simulink model "powertrain_model"  (R2025a)
settings: Solver=ode23tb  StartTime=0.0  StopTime=simlength  FixedStep=tc  MaxStep=tc
values from neighbouring files (symbols this model uses):
  angle_error = angle_error_deg/180*pi    (= 0)    [init_model.m]
  CTRPIFF_CLIP_RELEASE = 0.001    [init_model.m]
  dead_time = dead_time_INV    (= 4.2e-07)    [init_model.m]
  dead_time_INV = 0.42e-6    (= 4.2e-07)    [init_model.m]
  DThs_init = 0    [init_model.m]
  emf_fb_p = 0.2    [init_model.m]
  emf_fb_p_ccaller_1 = emf_fb_p    (= 0.2)    [init_model.m]
  emf_fb_p_ccaller_2 = emf_fb_p    (= 0.2)    [init_model.m]
  emf_p = emf_fb_p*4/10    (= 0.08)    [init_model.m]
  emf_p_ccaller_1 = emf_fb_p_ccaller_1*4/10    (= 0.08)    [init_model.m]
  emf_p_ccaller_2 = emf_fb_p_ccaller_2*4/10    (= 0.08)    [init_model.m]
  fPWM_INV = 25e3    (= 25000)    [init_model.m]
  g0_reference_flt = fcut_reference_flt * ts_inv * 2*pi    (= 0.00100530964915)    [init_model.m]
  g1_reference_flt = 1 - g0_reference_flt    (= 0.998994690351)    [init_model.m]
  id_ref_if_pu = iload_rms_ref*sqrt(2)/ibez    [init_model.m]
  kalman_omega = kw    [init_model.m]
  kalman_theta = kg    [init_model.m]
  kg = K(1)    [init_model.m]
  ki_id = 2    [analysis_cc.m]    (also in init_model.m = 9)
  ki_iq = 9    [init_model.m]
  ki_w = 1    [init_model.m]
  kp_id = 0.15    [analysis_cc.m]    (also in init_model.m = 0.25)
  kp_iq = 0.2    [init_model.m]
  kp_w = 1    [init_model.m]
  kw = K(2)    [init_model.m]
  luenberger_l1 = Klo(1)    [init_model.m]
  luenberger_l2 = Klo(2)    [init_model.m]
  luenberger_l3 = Klo(3)    [init_model.m]
  motorc_m_scale = 2/3*Vdc_bez/ubez    [init_model.m]
  number_of_cells = 100    [init_model.m]
  omega_flt_fcut = 10    [init_model.m]
  omega_flt_g0 = omega_flt_fcut * ts_inv * 2*pi    (= 0.00251327412287)    [init_model.m]
  omega_flt_g1 = 1 - omega_flt_g0    (= 0.997486725877)    [init_model.m]
  omega_ref_if_pu = 1200*2*pi/omega_bez    [init_model.m]
  phase_compensation_omega = 0    [init_model.m]
  pwm_out_lim = 1    [init_model.m]
  Q = 10    [init_model.m]
  q1Kalman = ts_inv^2    (= 1.6e-09)    [init_model.m]
  q2Kalman = ts_inv^1    (= 4e-05)    [init_model.m]
  q3Kalman = 0    [init_model.m]
  rKalman = 1    [init_model.m]
  Tambient = 1    [init_model.m]
  tc = ts_inv/200    (= 2e-07)    [init_model.m]
  time_init = 0.025    [init_model.m]
  torque_ref = 64/ibez*torque_mode    [init_model.m]
  ts_inv = 1/fPWM_INV    (= 4e-05)    [init_model.m]
  tsample = ts_inv    (= 4e-05)    [init_model.m]
  u_flt_g0 = u_flt_fcut * ts_inv * 2*pi    (= 0.904778684234)    [init_model.m]
  u_flt_g1 = 1 - u_flt_g0    (= 0.0952213157661)    [init_model.m]
  Vdc_bez = 400    [init_model.m]
undefined symbols (not defined in the file or in its folder): b, ibez, Jm, Jm_norm, Ld_norm, Lq_norm, Ls_norm, magnitude, omega_bez, psi_bez, psi_m, psi_m_norm, R_RLload, Rload_eq, Rs_norm, tau_bez, weigth
libraries: fl_lib x100, nesl_utility x84, ee_lib x11, cstblocks x4, lithium_ion_cell_lib x1, simulink x1, pmsm_uvw_with_harmonics_lib x1, pmsm_spatial_harmonics_uvw_lib x1, flexshaft_lib x1
(part 3 of 6)

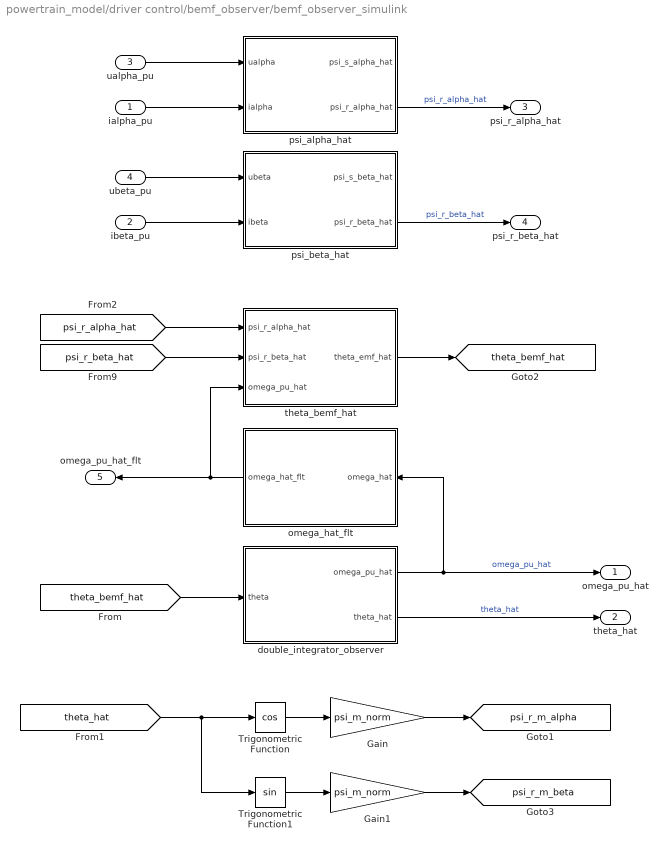
== system powertrain_model/driver control/bemf_observer/bemf_observer_simulink ==
  ialpha_pu : Inport
  ibeta_pu : Inport  Port=2
  ualpha_pu : Inport  Port=3
  ubeta_pu : Inport  Port=4
  Gain : Gain  Gain=psi_m_norm
  Gain1 : Gain  Gain=psi_m_norm
  Trigonometric Function : Trigonometry  Operator=cos
  Trigonometric Function1 : Trigonometry
  double_integrator_observer : Subsystem
  omega_hat_flt : Subsystem
  psi_alpha_hat : Subsystem
  psi_beta_hat : Subsystem
  theta_bemf_hat : Subsystem
  omega_pu_hat : Outport
  theta_hat : Outport  Port=2
  psi_r_alpha_hat : Outport  Port=3
  psi_r_beta_hat : Outport  Port=4
  omega_pu_hat_flt : Outport  Port=5
  tag scope: psi_r_m_alpha=global, psi_r_m_beta=global, theta_bemf_hat=global
  wires:
  omega_hat_flt/1(omega_hat_flt) -> omega_pu_hat_flt/1, theta_bemf_hat/3(omega_pu_hat)
  psi_alpha_hat/2(psi_r_alpha_hat) -> psi_r_alpha_hat/1  "psi_r_alpha_hat"
  double_integrator_observer/1(omega_pu_hat) -> omega_pu_hat/1, omega_hat_flt/1(omega_hat)  "omega_pu_hat"
  double_integrator_observer/2(theta_hat) -> theta_hat/1  "theta_hat"
  psi_beta_hat/2(psi_r_beta_hat) -> psi_r_beta_hat/1  "psi_r_beta_hat"
  [theta_bemf_hat] -> double_integrator_observer/1(theta)
  theta_bemf_hat/1(theta_emf_hat) -> [theta_bemf_hat]
  Gain1/1 -> [psi_r_m_beta]
  Gain/1 -> [psi_r_m_alpha]
  [theta_hat] -> Trigonometric Function1/1, Trigonometric Function/1
  ubeta_pu/1 -> psi_beta_hat/1(ubeta)
  ualpha_pu/1 -> psi_alpha_hat/1(ualpha)
  ibeta_pu/1 -> psi_beta_hat/2(ibeta)
  ialpha_pu/1 -> psi_alpha_hat/2(ialpha)
  Trigonometric Function1/1 -> Gain1/1
  Trigonometric Function/1 -> Gain/1
  [psi_r_alpha_hat] -> theta_bemf_hat/1(psi_r_alpha_hat)
  [psi_r_beta_hat] -> theta_bemf_hat/2(psi_r_beta_hat)

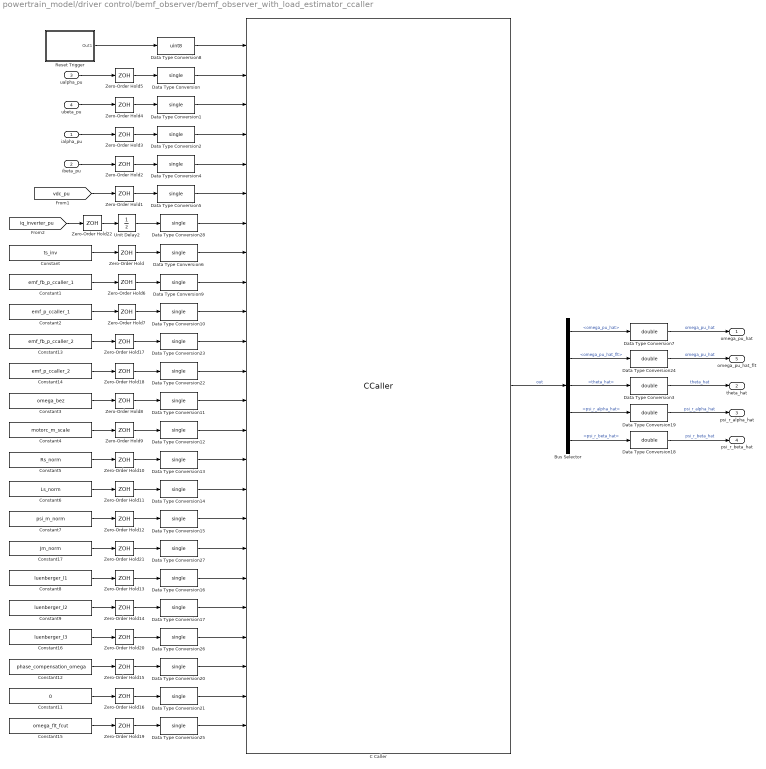
== system powertrain_model/driver control/bemf_observer/bemf_observer_with_load_estimator_ccaller ==
  ialpha_pu : Inport
  ibeta_pu : Inport  Port=2
  ualpha_pu : Inport  Port=3
  ubeta_pu : Inport  Port=4
  Bus Selector : BusSelector  OutputSignals=omega_pu_hat,omega_pu_hat_flt,theta_hat,psi_r_alpha_hat,psi_r_beta_hat
  C Caller : CCaller  FunctionName=bemf_obsv_load_est_process_simulink  PortSpecificationStruct="%)30     .    (\"P   8    (     @         %    \"    !D    !     0         %  0 \"0    $    _    07)G3F%M90  4&]R=$YA;64 4V-O<&4     26YD97@     5'EP90      4VEZ90      27-';&]B86P   X    P    !@    @    $          4    (     0    ,    !         !   P!O=70 #@   #     &    \"     0         !0    @    !     P    $         $  # &]U=  .    .     8    (    !          %    \"     $    &     0         0  ...(+14838 chars)"  SampleTime=ts_inv
  Constant : Constant  Value=ts_inv
  Constant1 : Constant  Value=emf_fb_p_ccaller_1
  Constant11 : Constant  Value=0
  Constant12 : Constant  Value=phase_compensation_omega  VectorParams1D=off
  Constant13 : Constant  Value=emf_fb_p_ccaller_2
  Constant14 : Constant  Value=emf_p_ccaller_2
  Constant15 : Constant  Value=omega_flt_fcut
  Constant16 : Constant  Value=luenberger_l3
  Constant17 : Constant  Value=Jm_norm
  Constant2 : Constant  Value=emf_p_ccaller_1
  Constant3 : Constant  Value=omega_bez
  Constant4 : Constant  Value=motorc_m_scale
  Constant5 : Constant  Value=Rs_norm
  Constant6 : Constant  Value=Ls_norm
  Constant7 : Constant  Value=psi_m_norm
  Constant8 : Constant  Value=luenberger_l1
  Constant9 : Constant  Value=luenberger_l2
  Data Type Conversion{,1..2,4..6,9..17,20..23,25..28} (23 alike) : DataTypeConversion  OutDataTypeStr=single  SaturateOnIntegerOverflow=off  RndMeth=Floor
  Data Type Conversion{3,7,18..19,24} (5 alike) : DataTypeConversion  OutDataTypeStr=double  SaturateOnIntegerOverflow=off  RndMeth=Floor
  Data Type Conversion8 : DataTypeConversion  OutDataTypeStr=uint8  SaturateOnIntegerOverflow=off  RndMeth=Floor
  Reset Trigger : Subsystem
  Unit Delay2 : UnitDelay  SampleTime=ts_inv  HasFrameUpgradeWarning=on
  Zero-Order Hold{,1..22} (23 alike) : ZeroOrderHold  SampleTime=ts_inv
  omega_pu_hat : Outport
  theta_hat : Outport  Port=2
  psi_r_alpha_hat : Outport  Port=3
  psi_r_beta_hat : Outport  Port=4
  omega_pu_hat_flt : Outport  Port=5
  wires:
  Data Type Conversion5/1 -> C Caller/6
  Data Type Conversion/1 -> C Caller/2
  Data Type Conversion1/1 -> C Caller/3
  Data Type Conversion4/1 -> C Caller/5
  Data Type Conversion2/1 -> C Caller/4
  Zero-Order Hold/1 -> Data Type Conversion6/1
  Zero-Order Hold5/1 -> Data Type Conversion/1
  Zero-Order Hold4/1 -> Data Type Conversion1/1
  Zero-Order Hold3/1 -> Data Type Conversion2/1
  Zero-Order Hold2/1 -> Data Type Conversion4/1
  Zero-Order Hold1/1 -> Data Type Conversion5/1
  [vdc_pu] -> Zero-Order Hold1/1
  Constant/1 -> Zero-Order Hold/1
  ualpha_pu/1 -> Zero-Order Hold5/1
  ialpha_pu/1 -> Zero-Order Hold3/1
  ubeta_pu/1 -> Zero-Order Hold4/1
  ibeta_pu/1 -> Zero-Order Hold2/1
  Reset Trigger/1(Out1) -> Data Type Conversion8/1
  Data Type Conversion8/1 -> C Caller/1
  Zero-Order Hold6/1 -> Data Type Conversion9/1
  Zero-Order Hold7/1 -> Data Type Conversion10/1
  Zero-Order Hold8/1 -> Data Type Conversion11/1
  Zero-Order Hold9/1 -> Data Type Conversion12/1
  Zero-Order Hold10/1 -> Data Type Conversion13/1
  Zero-Order Hold11/1 -> Data Type Conversion14/1
  Zero-Order Hold12/1 -> Data Type Conversion15/1
  Zero-Order Hold13/1 -> Data Type Conversion16/1
  Zero-Order Hold14/1 -> Data Type Conversion17/1
  Constant3/1 -> Zero-Order Hold8/1
  Constant4/1 -> Zero-Order Hold9/1
  Constant5/1 -> Zero-Order Hold10/1
  Constant8/1 -> Zero-Order Hold13/1
  Constant9/1 -> Zero-Order Hold14/1
  Constant6/1 -> Zero-Order Hold11/1
  Constant7/1 -> Zero-Order Hold12/1
  C Caller/1 -> Bus Selector/1  "out"
  Data Type Conversion7/1 -> omega_pu_hat/1  "omega_pu_hat"
  Data Type Conversion3/1 -> theta_hat/1  "theta_hat"
  Data Type Conversion19/1 -> psi_r_alpha_hat/1  "psi_r_alpha_hat"
  Data Type Conversion18/1 -> psi_r_beta_hat/1  "psi_r_beta_hat"
  Constant1/1 -> Zero-Order Hold6/1
  Constant2/1 -> Zero-Order Hold7/1
  Constant12/1 -> Zero-Order Hold15/1
  Zero-Order Hold15/1 -> Data Type Conversion20/1
  Zero-Order Hold16/1 -> Data Type Conversion21/1
  Constant11/1 -> Zero-Order Hold16/1
  Constant14/1 -> Zero-Order Hold18/1
  Constant13/1 -> Zero-Order Hold17/1
  Zero-Order Hold18/1 -> Data Type Conversion22/1
  Zero-Order Hold17/1 -> Data Type Conversion23/1
  Data Type Conversion24/1 -> omega_pu_hat_flt/1  "omega_pu_hat"
  Constant15/1 -> Zero-Order Hold19/1
  Zero-Order Hold19/1 -> Data Type Conversion25/1
  Bus Selector/5 -> Data Type Conversion18/1  "<psi_r_beta_hat>"
  Bus Selector/4 -> Data Type Conversion19/1  "<psi_r_alpha_hat>"
  Bus Selector/3 -> Data Type Conversion3/1  "<theta_hat>"
  Bus Selector/2 -> Data Type Conversion24/1  "<omega_pu_hat_flt>"
  Bus Selector/1 -> Data Type Conversion7/1  "<omega_pu_hat>"
  Constant16/1 -> Zero-Order Hold20/1
  Zero-Order Hold20/1 -> Data Type Conversion26/1
  Constant17/1 -> Zero-Order Hold21/1
  Zero-Order Hold21/1 -> Data Type Conversion27/1
  Data Type Conversion6/1 -> C Caller/8
  Data Type Conversion9/1 -> C Caller/9
  Data Type Conversion10/1 -> C Caller/10
  Data Type Conversion23/1 -> C Caller/11
  Data Type Conversion22/1 -> C Caller/12
  Data Type Conversion11/1 -> C Caller/13
  Data Type Conversion12/1 -> C Caller/14
  Data Type Conversion13/1 -> C Caller/15
  Data Type Conversion14/1 -> C Caller/16
  Data Type Conversion15/1 -> C Caller/17
  Data Type Conversion27/1 -> C Caller/18
  Data Type Conversion16/1 -> C Caller/19
  Data Type Conversion17/1 -> C Caller/20
  Data Type Conversion26/1 -> C Caller/21
  Data Type Conversion20/1 -> C Caller/22
  Data Type Conversion21/1 -> C Caller/23
  Data Type Conversion25/1 -> C Caller/24
  [iq_inverter_pu] -> Zero-Order Hold22/1
  Zero-Order Hold22/1 -> Unit Delay2/1
  Data Type Conversion28/1 -> C Caller/7
  Unit Delay2/1 -> Data Type Conversion28/1

== system powertrain_model/driver control/bemf_observer/u_alpha_flt ==
  u : Inport
  Gain3 : Gain  Gain=u_flt_g1
  Gain6 : Gain  Gain=u_flt_g0
  Sum : Sum  Inputs=|++
  Unit Delay1 : UnitDelay  SampleTime=ts_inv  HasFrameUpgradeWarning=on
  u_flt : Outport  VectorParamsAs1DForOutWhenUnconnected=off
  wires:
  Sum/1 -> u_flt/1, Unit Delay1/1
  Gain3/1 -> Sum/2
  Unit Delay1/1 -> Gain3/1
  u/1 -> Gain6/1
  Gain6/1 -> Sum/1

== system powertrain_model/driver control/bemf_observer/u_beta_flt ==
  u : Inport
  Gain3 : Gain  Gain=u_flt_g1
  Gain6 : Gain  Gain=u_flt_g0
  Sum : Sum  Inputs=|++
  Unit Delay1 : UnitDelay  SampleTime=ts_inv  HasFrameUpgradeWarning=on
  u_flt : Outport  VectorParamsAs1DForOutWhenUnconnected=off
  wires:
  Gain6/1 -> Sum/1
  u/1 -> Gain6/1
  Unit Delay1/1 -> Gain3/1
  Gain3/1 -> Sum/2
  Sum/1 -> Unit Delay1/1, u_flt/1

== system powertrain_model/driver control/current_ctrl/current_transformation ==
  u : Inport
  v : Inport  Port=2
  w : Inport  Port=3
  phase : Inport  Port=4
  alphabeta2dq : MATLAB Function  TreatAsAtomicUnit=on  SystemSampleTime=ts_inv
  uvw2alphabeta : MATLAB Function  TreatAsAtomicUnit=on  SystemSampleTime=ts_inv
  tag scope: i_alpha_inverter_pu=global, i_beta_inverter_pu=global, id_inverter_pu=global, iq_inverter_pu=global
  wires:
  u/1 -> uvw2alphabeta/1(u)
  uvw2alphabeta/1(alpha) -> [i_alpha_inverter_pu], alphabeta2dq/1(alpha)  "ialpha_if_pu"
  uvw2alphabeta/2(beta) -> [i_beta_inverter_pu], alphabeta2dq/2(beta)  "ibeta_if_pu"
  v/1 -> uvw2alphabeta/2(v)
  w/1 -> uvw2alphabeta/3(w)
  alphabeta2dq/1(d) -> [id_inverter_pu]
  alphabeta2dq/2(q) -> [iq_inverter_pu]
  phase/1 -> alphabeta2dq/3(phase)

== system powertrain_model/driver control/current_ctrl/rotor_phase_selection ==
  Scope : Scope  NumInputPorts=2
      settings: ActiveDisplayYMinimum=-3.92698  ActiveDisplayYMaximum=3.92699
  Switch1 : Switch  Criteria=u2 > Threshold  Threshold=0.1  SaturateOnIntegerOverflow=off  InputSameDT=off
  Switch2 : Switch  Criteria=u2 > Threshold  Threshold=0.1  SaturateOnIntegerOverflow=off  InputSameDT=off
  Variant Source : VariantSource  VariantControls={use_gyro_model == 1, use_gyro_model == 0}
  Variant Source1 : VariantSource  VariantControls={use_I_F_control == 1, use_I_F_control == 0}
  Variant Source2 : VariantSource  VariantControls={1==0, 1==1}
  theta_ctrl : Outport
  wires:
  [omega_pu_hat] -> Switch1/2
  [theta_pmsm] -> Switch1/3
  [theta_hat] -> Switch1/1
  Switch2/1 -> Variant Source/1
  Switch1/1 -> Variant Source/2
  Variant Source/1 -> Variant Source1/2
  [theta_ref_if_control] -> Variant Source1/1
  [theta_hat] -> Switch2/1
  [theta_pmsm] -> Switch2/3
  [omega_pu_hat] -> Switch2/2
  [theta_hat] -> Variant Source2/2, Scope/2  "theta_hat"
  [theta_pmsm] -> Scope/1, Variant Source2/1  "theta_pmsm"
  [theta_hat] -> theta_ctrl/1

== system powertrain_model/driver control/current_ctrl/sample_hold_normalization ==
  iu : Inport
  iv : Inport  Port=2
  iw : Inport  Port=3
  Gain : Gain  Gain=1/ibez
  Gain1 : Gain  Gain=1/ibez
  Gain2 : Gain  Gain=1/ibez
  LTI System : cstblocks/LTI System  sys=cm_tf  IC=[]  PadeOrder=0
  LTI System1 : cstblocks/LTI System  sys=cm_tf  IC=[]  PadeOrder=0
  LTI System2 : cstblocks/LTI System  sys=cm_tf  IC=[]  PadeOrder=0
  Unit Delay : UnitDelay  SampleTime=ts_inv  HasFrameUpgradeWarning=on
  Unit Delay1 : UnitDelay  SampleTime=ts_inv  HasFrameUpgradeWarning=on
  Unit Delay4 : UnitDelay  SampleTime=ts_inv  HasFrameUpgradeWarning=on
  Zero-Order Hold : ZeroOrderHold  SampleTime=ts_inv
  Zero-Order Hold1 : ZeroOrderHold  SampleTime=ts_inv
  Zero-Order Hold2 : ZeroOrderHold  SampleTime=ts_inv
  iu_pu : Outport
  iv_pu : Outport  Port=2
  iw_pu : Outport  Port=3
  wires:
  Zero-Order Hold/1 -> Unit Delay/1
  Zero-Order Hold2/1 -> Unit Delay4/1
  Zero-Order Hold1/1 -> Unit Delay1/1
  Gain1/1 -> iv_pu/1
  Gain2/1 -> iw_pu/1
  Gain/1 -> iu_pu/1
  iu/1 -> LTI System/1
  iv/1 -> LTI System1/1
  iw/1 -> LTI System2/1
  LTI System1/1 -> Zero-Order Hold1/1
  LTI System/1 -> Zero-Order Hold/1
  LTI System2/1 -> Zero-Order Hold2/1
  Unit Delay4/1 -> Gain2/1
  Unit Delay1/1 -> Gain1/1
  Unit Delay/1 -> Gain/1

== system powertrain_model/driver control/current_ctrl/vector_current_ctrl ==
  iq_ref : Inport
  id_ref : Inport  Port=2
  MTPA : Subsystem
      settings: PortSchema="{\"entries\":[{\"content\":{\"sides\":[{\"content\":{\"connectorIds\":[\"In1\"]},\"type\":\"ConnectorPlacement.EquallySpacedRectSide\",\"uuid\":\"b7b50820-32cf-4b06-b710-c36db40508fb\"},{\"content\":{\"connectorIds\":[\"Out1\"],\"side\":\"RIGHT\"},\"type\":\"ConnectorPlacement.EquallySpacedRectSide\",\"uuid\":\"9680176d-6365-4ae4-8330-83815ae14f93\"},{\"content\":{\"connectorIds\":[\"In2\"],\"side\":\"TOP\"},\"type\":\"ConnectorPlacement.EquallySpacedRectSide\",\"uuid\":\"503d8594-1c43-4fac-b8a6-77f5afdeeec1\"}]},\"type\":\"ConnectorPlacement.EquallySpacedConnector\",\"uuid\":\"c97785bf-1f92-4066-ba86-64cef6027105\"}],\"packageUris\":[\"http://schema.mathworks.com/mf0/Connector/R2020b\"],\"version\":\"1.0\"}"
  Variant Source : VariantSource  ShowConditionOnBlock=on  VariantControls={use_cc_ccaller == 1, use_cc_simulink == 1}
  Variant Source1 : VariantSource  ShowConditionOnBlock=on  VariantControls={use_cc_ccaller == 1, use_cc_simulink == 1}
  dq_vector_pi : Subsystem
  dq_vector_pi_ccaller : Subsystem
  id_ref_pu/id_pu : Scope  NumInputPorts=2
      settings: SampleTime=tc  ActiveDisplayYMinimum=-1.3102981633371098  ActiveDisplayYMaximum=1.2629412816594339
  iq_ref_pu/iq_pu : Scope  NumInputPorts=2
      settings: SampleTime=tc  ActiveDisplayYMinimum=-0.14495  ActiveDisplayYMaximum=1.30456  DataLoggingVariableName=ScopeData2
  ud : Outport
  uq : Outport  Port=2
  tag scope: id_ref_inverter_pu=global, iq_ref_inverter_pu=global, ud_inverter_pu=global, uq_inverter_pu=global
  wires:
  [iq_inverter_pu] -> dq_vector_pi/3(iq), iq_ref_pu/iq_pu/2, dq_vector_pi_ccaller/3(iq)  "iq_inverter_pu"
  [id_inverter_pu] -> dq_vector_pi/1(id), dq_vector_pi_ccaller/1(id), id_ref_pu/id_pu/2  "id_inverter_pu"
  MTPA/1(id_ref) -> dq_vector_pi/2(id_ref), dq_vector_pi_ccaller/2(id_ref), [id_ref_inverter_pu], id_ref_pu/id_pu/1  "id_ref"
  id_ref/1 -> MTPA/2(id_ref_ext)
  Variant Source/1 -> [ud_inverter_pu], ud/1
  dq_vector_pi_ccaller/1(ud_ctrl_out) -> Variant Source/1
  dq_vector_pi_ccaller/2(uq_ctrl_out) -> Variant Source1/1
  Variant Source1/1 -> [uq_inverter_pu], uq/1
  dq_vector_pi/1(ctrl_d_u) -> Variant Source/2
  dq_vector_pi/2(ctrl_q_u) -> Variant Source1/2
  iq_ref/1 -> MTPA/1(iq_ref), dq_vector_pi/4(iq_ref), [iq_ref_inverter_pu], iq_ref_pu/iq_pu/1, dq_vector_pi_ccaller/4(iq_ref)  "iq_ref"

== system powertrain_model/driver control/i//f references/filter_pt1 ==
  input : Inport
  Gain3 : Gain  Gain=g1_reference_flt
  Gain6 : Gain  Gain=g0_reference_flt
  Sum : Sum  Inputs=|++
  Unit Delay1 : UnitDelay  SampleTime=ts_inv  HasFrameUpgradeWarning=on
  output : Outport  VectorParamsAs1DForOutWhenUnconnected=off
  wires:
  Gain6/1 -> Sum/1
  input/1 -> Gain6/1
  Unit Delay1/1 -> Gain3/1
  Gain3/1 -> Sum/2
  Sum/1 -> Unit Delay1/1, output/1

== system powertrain_model/driver control/i//f references/filter_pt2 ==
  input : Inport
  Gain3 : Gain  Gain=g1_reference_flt
  Gain6 : Gain  Gain=g0_reference_flt
  Sum : Sum  Inputs=|++
  Unit Delay1 : UnitDelay  SampleTime=ts_inv  HasFrameUpgradeWarning=on
  output : Outport  VectorParamsAs1DForOutWhenUnconnected=off
  wires:
  Sum/1 -> output/1, Unit Delay1/1
  Gain3/1 -> Sum/2
  Unit Delay1/1 -> Gain3/1
  input/1 -> Gain6/1
  Gain6/1 -> Sum/1

== system powertrain_model/driver control/speed_loop/Speed control ==
  Rotor speed : Inport
  Speed ref : Inport  Port=2
  1/Ti : Gain  Gain=kp_w  SaturateOnIntegerOverflow=on  OutDataTypeStr=Inherit: Same as input  ParamDataTypeStr=Inherit: Same as input
  Saturation : Saturate  UpperLimit=1.1  LowerLimit=-1.1
  Sum1 : Sum  Inputs=+++  SaturateOnIntegerOverflow=on
  Sum2 : Sum  Inputs=-+  SaturateOnIntegerOverflow=on
  Sum3 : Sum  Inputs=-+  SaturateOnIntegerOverflow=on
  Unit Delay4 : UnitDelay  SampleTime=ts_inv  HasFrameUpgradeWarning=on
  kp : Gain  Gain=ki_w*ts_inv  SaturateOnIntegerOverflow=on  OutDataTypeStr=Inherit: Same as input  ParamDataTypeStr=Inherit: Same as input
  torque_ref : Outport
  wires:
  1/Ti/1 -> Sum1/1, Sum3/1
  kp/1 -> Sum1/2
  Sum3/1 -> Unit Delay4/1
  Unit Delay4/1 -> Sum1/3
  Speed ref/1 -> Sum2/2
  Rotor speed/1 -> Sum2/1
  Sum2/1 -> kp/1, 1/Ti/1
  Sum1/1 -> Saturation/1
  Saturation/1 -> torque_ref/1, Sum3/2

== system powertrain_model/driver control/torque_reference_generator/reference_d_flt ==
  input : Inport
  Gain3 : Gain  Gain=g1_reference_flt
  Gain6 : Gain  Gain=g0_reference_flt
  Sum : Sum  Inputs=|++
  Unit Delay1 : UnitDelay  SampleTime=ts_inv  HasFrameUpgradeWarning=on
  output : Outport  VectorParamsAs1DForOutWhenUnconnected=off
  wires:
  Gain6/1 -> Sum/1
  input/1 -> Gain6/1
  Unit Delay1/1 -> Gain3/1
  Gain3/1 -> Sum/2
  Sum/1 -> Unit Delay1/1, output/1

== system powertrain_model/driver control/torque_reference_generator/reference_q_flt ==
  input : Inport
  Gain3 : Gain  Gain=g1_reference_flt
  Gain6 : Gain  Gain=g0_reference_flt
  Sum : Sum  Inputs=|++
  Unit Delay1 : UnitDelay  SampleTime=ts_inv  HasFrameUpgradeWarning=on
  output : Outport  VectorParamsAs1DForOutWhenUnconnected=off
  wires:
  Sum/1 -> output/1, Unit Delay1/1
  Gain3/1 -> Sum/2
  Unit Delay1/1 -> Gain3/1
  input/1 -> Gain6/1
  Gain6/1 -> Sum/1

== system powertrain_model/inverter/Gyro based inverter/gyro1 ==
  m : Inport
  Controlled Current Source : fl_lib/Electrical/Electrical Sources/Controlled Current Source
  Controlled Voltage Source : fl_lib/Electrical/Electrical Sources/Controlled Voltage Source
  Current Sensor : fl_lib/Electrical/Electrical Sensors/Current Sensor
  PS Product : fl_lib/Physical Signals/Functions/PS Product
  PS Product1 : fl_lib/Physical Signals/Functions/PS Product
  Simulink-PS Converter : nesl_utility/Simulink-PS Converter  PhysicalDomain=network_engine_domain  SubClassName=ps_input  LeftPortType=input  RightPortType=output  PseudoPeriodic=off  Frequencies=[]  NoiseDistribution=none  NoiseParameters=[]  Unit=1  AffineConversion=on  FilteringAndDerivatives=provide  SimscapeFilterOrder=1  InputFilterTimeConstant=0.001  UdotUserProvided=0
  Voltage Sensor : fl_lib/Electrical/Electrical Sensors/Voltage Sensor
  uin+ : PMIOPort  Side=Left
  uin- : PMIOPort  Port=2  Side=Left
  uout+ : PMIOPort  Port=3  Side=Right
  uout- : PMIOPort  Port=4  Side=Right
  wires:
  m/1 -> Simulink-PS Converter/1
  connections:
  Voltage Sensor/RConn2 -- Controlled Current Source/LConn1 -- uin-/RConn1
  Voltage Sensor/LConn1 -- Controlled Current Source/RConn2 -- uin+/RConn1
  Controlled Voltage Source/LConn1 -- Current Sensor/LConn1
  Controlled Voltage Source/RConn2 -- uout-/RConn1
  Current Sensor/RConn2 -- uout+/RConn1
  Simulink-PS Converter/RConn1 -- PS Product/LConn1 -- PS Product1/LConn2
  Voltage Sensor/RConn1 -- PS Product/LConn2
  PS Product1/RConn1 -- Controlled Current Source/RConn1
  PS Product/RConn1 -- Controlled Voltage Source/RConn1
  Current Sensor/RConn1 -- PS Product1/LConn1

== system powertrain_model/inverter/Gyro based inverter/gyro2 ==
  m : Inport
  Controlled Current Source : fl_lib/Electrical/Electrical Sources/Controlled Current Source
  Controlled Voltage Source : fl_lib/Electrical/Electrical Sources/Controlled Voltage Source
  Current Sensor : fl_lib/Electrical/Electrical Sensors/Current Sensor
  PS Product : fl_lib/Physical Signals/Functions/PS Product
  PS Product1 : fl_lib/Physical Signals/Functions/PS Product
  Simulink-PS Converter : nesl_utility/Simulink-PS Converter  PhysicalDomain=network_engine_domain  SubClassName=ps_input  LeftPortType=input  RightPortType=output  PseudoPeriodic=off  Frequencies=[]  NoiseDistribution=none  NoiseParameters=[]  Unit=1  AffineConversion=on  FilteringAndDerivatives=provide  SimscapeFilterOrder=1  InputFilterTimeConstant=0.001  UdotUserProvided=0
  Voltage Sensor : fl_lib/Electrical/Electrical Sensors/Voltage Sensor
  uin+ : PMIOPort  Side=Left
  uin- : PMIOPort  Port=2  Side=Left
  uout+ : PMIOPort  Port=3  Side=Right
  uout- : PMIOPort  Port=4  Side=Right
  wires:
  m/1 -> Simulink-PS Converter/1
  connections:
  Current Sensor/RConn1 -- PS Product1/LConn1
  PS Product/RConn1 -- Controlled Voltage Source/RConn1
  PS Product1/RConn1 -- Controlled Current Source/RConn1
  Voltage Sensor/RConn1 -- PS Product/LConn2
  PS Product1/LConn2 -- PS Product/LConn1 -- Simulink-PS Converter/RConn1
  Current Sensor/RConn2 -- uout+/RConn1
  Controlled Voltage Source/RConn2 -- uout-/RConn1
  Controlled Voltage Source/LConn1 -- Current Sensor/LConn1
  uin+/RConn1 -- Controlled Current Source/RConn2 -- Voltage Sensor/LConn1
  uin-/RConn1 -- Controlled Current Source/LConn1 -- Voltage Sensor/RConn2

== system powertrain_model/inverter/Gyro based inverter/gyro3 ==
  m : Inport
  Controlled Current Source : fl_lib/Electrical/Electrical Sources/Controlled Current Source
  Controlled Voltage Source : fl_lib/Electrical/Electrical Sources/Controlled Voltage Source
  Current Sensor : fl_lib/Electrical/Electrical Sensors/Current Sensor
  PS Product : fl_lib/Physical Signals/Functions/PS Product
  PS Product1 : fl_lib/Physical Signals/Functions/PS Product
  Simulink-PS Converter : nesl_utility/Simulink-PS Converter  PhysicalDomain=network_engine_domain  SubClassName=ps_input  LeftPortType=input  RightPortType=output  PseudoPeriodic=off  Frequencies=[]  NoiseDistribution=none  NoiseParameters=[]  Unit=1  AffineConversion=on  FilteringAndDerivatives=provide  SimscapeFilterOrder=1  InputFilterTimeConstant=0.001  UdotUserProvided=0
  Voltage Sensor : fl_lib/Electrical/Electrical Sensors/Voltage Sensor
  uin+ : PMIOPort  Side=Left
  uin- : PMIOPort  Port=2  Side=Left
  uout+ : PMIOPort  Port=3  Side=Right
  uout- : PMIOPort  Port=4  Side=Right
  wires:
  m/1 -> Simulink-PS Converter/1
  connections:
  Voltage Sensor/RConn2 -- Controlled Current Source/LConn1 -- uin-/RConn1
  Voltage Sensor/LConn1 -- Controlled Current Source/RConn2 -- uin+/RConn1
  Controlled Voltage Source/LConn1 -- Current Sensor/LConn1
  Controlled Voltage Source/RConn2 -- uout-/RConn1
  Current Sensor/RConn2 -- uout+/RConn1
  Simulink-PS Converter/RConn1 -- PS Product/LConn1 -- PS Product1/LConn2
  Voltage Sensor/RConn1 -- PS Product/LConn2
  PS Product1/RConn1 -- Controlled Current Source/RConn1
  PS Product/RConn1 -- Controlled Voltage Source/RConn1
  Current Sensor/RConn1 -- PS Product1/LConn1

== system powertrain_model/inverter/MOS based inverter/inverter ==
  inverter_mosfet_leg_thermal : Subsystem
  inverter_without_mosfet_leg_thermal : Subsystem  Commented=on
  udc(+) : PMIOPort  Side=Left
  udc(-) : PMIOPort  Port=2  Side=Left
  u : PMIOPort  Port=3  Side=Right
  v : PMIOPort  Port=4  Side=Right
  w : PMIOPort  Port=5  Side=Right
  connections:
  udc(+)/RConn1 -- inverter_without_mosfet_leg_thermal/LConn1 -- inverter_mosfet_leg_thermal/LConn1
  inverter_mosfet_leg_thermal/RConn1 -- inverter_without_mosfet_leg_thermal/RConn1 -- u/RConn1
  inverter_mosfet_leg_thermal/RConn2 -- inverter_without_mosfet_leg_thermal/RConn2 -- v/RConn1
  w/RConn1 -- inverter_without_mosfet_leg_thermal/RConn3 -- inverter_mosfet_leg_thermal/RConn3
  udc(-)/RConn1 -- inverter_without_mosfet_leg_thermal/LConn2 -- inverter_mosfet_leg_thermal/LConn2

== system powertrain_model/inverter/MOS based inverter/sv_pwm ==
  ab : Inport
  Bus Selector : BusSelector  OutputSignals=da,db,dc
  Bus Selector1 : BusSelector  OutputSignals=ua,ub
  C Caller : CCaller  FunctionName=sv_pwm_process_simulink  PortSpecificationStruct="%)30     .    V @   8    (     @         %    \"     4    !     0         %  0 \"0    $    _    07)G3F%M90  4&]R=$YA;64 4V-O<&4     26YD97@     5'EP90      4VEZ90      27-';&]B86P   X    P    !@    @    $          4    (     0    ,    !         !   P!O=70 #@   #     &    \"     0         !0    @    !     P    $         $  # &]U=  .    .     8    (    !          %    \"     $    &     0         0   ...(+2669 chars)"  SampleTime=ts_inv
  Constant : Constant  Value=ts_inv
  Data Type Conversion1 : DataTypeConversion  OutDataTypeStr=double  SaturateOnIntegerOverflow=off  RndMeth=Floor
  Data Type Conversion15 : DataTypeConversion  OutDataTypeStr=single  SaturateOnIntegerOverflow=off  RndMeth=Floor
  Data Type Conversion16 : DataTypeConversion  OutDataTypeStr=single  SaturateOnIntegerOverflow=off  RndMeth=Floor
  Data Type Conversion17 : DataTypeConversion  OutDataTypeStr=uint32  SaturateOnIntegerOverflow=off  RndMeth=Floor
  Data Type Conversion18 : DataTypeConversion  OutDataTypeStr=single  SaturateOnIntegerOverflow=off  RndMeth=Floor
  Data Type Conversion2 : DataTypeConversion  OutDataTypeStr=double  SaturateOnIntegerOverflow=off  RndMeth=Floor
  Data Type Conversion3 : DataTypeConversion  OutDataTypeStr=double  SaturateOnIntegerOverflow=off  RndMeth=Floor
  Zero-Order Hold{,1..3} (4 alike) : ZeroOrderHold  SampleTime=ts_inv
  modulator : Subsystem
  modulator1 : Subsystem  Commented=on
  time_init : Step  Time=time_init  SampleTime=0
  firing_gates : Outport
  tag scope: mu_inverter=global, mv_inverter=global, mw_inverter=global
  wires:
  Data Type Conversion1/1 -> [mu_inverter], modulator/1(u)  "du"
  Zero-Order Hold/1 -> C Caller/1
  Zero-Order Hold2/1 -> C Caller/3
  Constant/1 -> Data Type Conversion16/1
  Bus Selector/1 -> Data Type Conversion1/1  "<da>"
  Data Type Conversion18/1 -> Zero-Order Hold/1
  Bus Selector/3 -> Data Type Conversion3/1  "<dc>"
  Data Type Conversion2/1 -> [mv_inverter], modulator/2(v)  "dv"
  Data Type Conversion16/1 -> Zero-Order Hold2/1
  Zero-Order Hold1/1 -> C Caller/2
  Data Type Conversion17/1 -> Zero-Order Hold3/1
  Zero-Order Hold3/1 -> C Caller/4
  Data Type Conversion15/1 -> Zero-Order Hold1/1
  C Caller/1 -> Bus Selector/1  "out"
  Bus Selector/2 -> Data Type Conversion2/1  "<db>"
  Data Type Conversion3/1 -> [mw_inverter], modulator/3(w)  "dw"
  modulator/1(firing_gates) -> firing_gates/1
  ab/1 -> Bus Selector1/1
  Bus Selector1/1 -> Data Type Conversion18/1  "<ua>"
  Bus Selector1/2 -> Data Type Conversion15/1  "<ub>"
  time_init/1 -> Data Type Conversion17/1

== system powertrain_model/inverter/MOS based inverter/threePhsModulator ==
  uab_pu : Inport
  Bus Creator1 : BusCreator  Inputs=2
  Bus Creator2 : BusCreator  Inputs=2
  Bus Creator3 : BusCreator  Inputs=3
  Bus Creator4 : BusCreator  Inputs=2
  Demux1 : Demux  Outputs=2
  Gain6 : Gain  Gain=1/sqrt(3)*2
  Gain7 : Gain  Gain=1/sqrt(3)*2
  Gain8 : Gain  Gain=1/sqrt(3)*2
  PWM generator 1 : Subsystem  mask{f=fPWM_INV, ph=0, m_up=1, m_low=-1, dead_time=dead_time, gate_voltage=15}
      mask prompts: f "Frequency"; ph "Phase"; m_up "Max Input Modulation Value"; m_low "Min Input Modulation Value"; dead_time "Dead Time"; gate_voltage "Gate Voltage"
  PWM generator 2 : Subsystem  mask{f=fPWM_INV, ph=0, m_up=1, m_low=-1, dead_time=dead_time, gate_voltage=15}
      mask prompts: f "Frequency"; ph "Phase"; m_up "Max Input Modulation Value"; m_low "Min Input Modulation Value"; dead_time "Dead Time"; gate_voltage "Gate Voltage"
  PWM generator 3 : Subsystem  mask{f=fPWM_INV, ph=0, m_up=1, m_low=-1, dead_time=dead_time, gate_voltage=15}
      mask prompts: f "Frequency"; ph "Phase"; m_up "Max Input Modulation Value"; m_low "Min Input Modulation Value"; dead_time "Dead Time"; gate_voltage "Gate Voltage"
  Sum : Sum  Inputs=|+-
  Sum1 : Sum  Inputs=|+-
  Sum2 : Sum  Inputs=|+-
  Third harmonic injecting : Subsystem
  du/dv/dw : Scope  NumInputPorts=3
      settings: SampleTime=ts_inv  ActiveDisplayYMinimum=-0.56429  ActiveDisplayYMaximum=0.52777
  uvw2alphabeta1 : MATLAB Function  TreatAsAtomicUnit=on  SystemSampleTime=ts_inv
  mout : Outport
  wires:
  uab_pu/1 -> Demux1/1
  Demux1/1 -> uvw2alphabeta1/1(alpha)
  Demux1/2 -> uvw2alphabeta1/2(beta)
  Third harmonic injecting/1(thind_H) -> Sum1/2, Sum/2, Sum2/2
  uvw2alphabeta1/1(u) -> Third harmonic injecting/1(m1), Sum/1  "ur"
  uvw2alphabeta1/2(v) -> Third harmonic injecting/2(m2), Sum1/1  "vr"
  uvw2alphabeta1/3(w) -> Sum2/1, Third harmonic injecting/3(m3)  "wr"
  Sum/1 -> Gain6/1
  Bus Creator3/1 -> mout/1
  PWM generator 1/1(m1) -> Bus Creator1/1  "gate_command_1"
  PWM generator 1/2(m2) -> Bus Creator1/2  "gate_command_2"
  Bus Creator1/1 -> Bus Creator3/1  "legA"
  PWM generator 2/2(m2) -> Bus Creator2/2  "gate_command_4"
  PWM generator 2/1(m1) -> Bus Creator2/1  "gate_command_3"
  PWM generator 3/1(m1) -> Bus Creator4/1  "gate_command_5"
  PWM generator 3/2(m2) -> Bus Creator4/2  "gate_command_6"
  Bus Creator2/1 -> Bus Creator3/2  "legB"
  Bus Creator4/1 -> Bus Creator3/3  "legC"
  Sum1/1 -> Gain7/1
  Sum2/1 -> Gain8/1
  Gain6/1 -> du/dv/dw/1, PWM generator 1/1(m_index)  "mu"
  Gain8/1 -> du/dv/dw/3, PWM generator 3/1(m_index)  "mw"
  Gain7/1 -> PWM generator 2/1(m_index), du/dv/dw/2  "mv"
